simulink model "fw_rc_mapping"  (R2026b)
settings: Solver=VariableStepAuto
undefined symbols (not defined in the file or in its folder): P, Ts
libraries: simulink x27
settings Model: Creator=aomar  LastModifiedBy=aomar

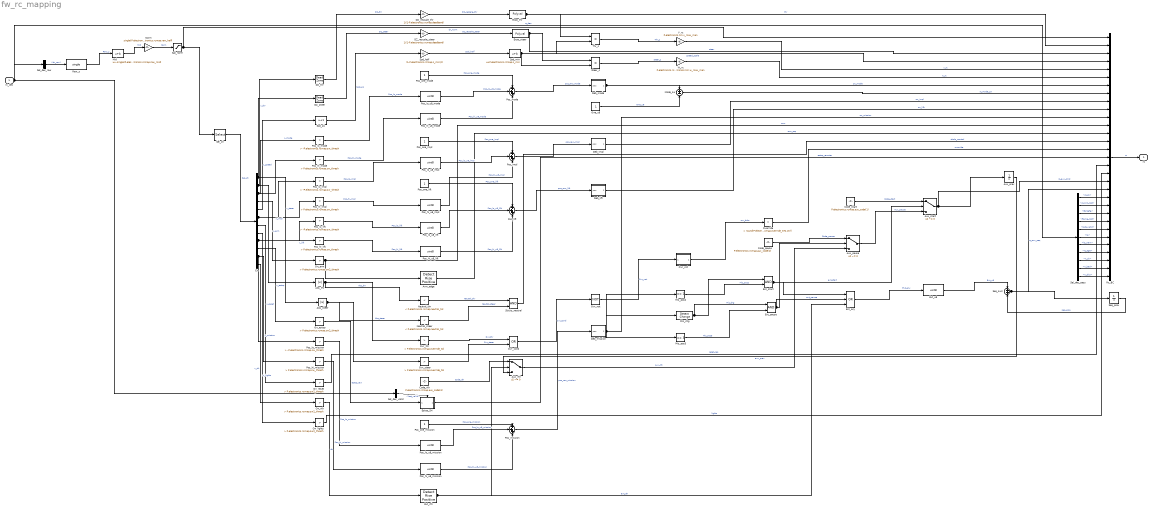
== system fw_rc_mapping ==
  rc_dec : Inport  SampleTime=Ts.ctrl
  Abs_steer : Abs  SaturateOnIntegerOverflow=off
  Abs_thr : Abs  SaturateOnIntegerOverflow=off
  Arm_edge : simulink/Logic and Bit Operations/Detect Rise Positive  vinit=0  OutDataTypeStr=boolean
  Aux_pause : Switch  Criteria=u2 ~= 0  SaturateOnIntegerOverflow=off  InputSameDT=off
  Aux_prev : UnitDelay  SampleTime=-1
  Aux_rth : Switch  Criteria=u2 ~= 0  SaturateOnIntegerOverflow=off  InputSameDT=off
  Aux_start : Switch  Criteria=u2 ~= 0  SaturateOnIntegerOverflow=off  InputSameDT=off
  Ch : Demux  Outputs=12
  Code_pause : Constant  Value=P.electronics.rcmap.aux_code(2)  OutDataTypeStr=uint8  SampleTime=-1
  Code_rth : Constant  Value=P.electronics.rcmap.aux_code(3)  OutDataTypeStr=uint8  SampleTime=-1
  Code_start : Constant  Value=P.electronics.rcmap.aux_code(1)  OutDataTypeStr=uint8  SampleTime=-1
  DZ_rescale_steer : Gain  Gain=1/(1-P.electronics.rcmap.deadband)
  DZ_rescale_thr : Gain  Gain=1/(1-P.electronics.rcmap.deadband)
  DZ_steer : DeadZone  LowerValue=-P.electronics.rcmap.deadband  UpperValue=P.electronics.rcmap.deadband
  DZ_thr : DeadZone  LowerValue=-P.electronics.rcmap.deadband  UpperValue=P.electronics.rcmap.deadband
  Deb_impl : Subsystem
  Deb_lift : Subsystem
  Deb_mission : Subsystem
  Deb_mode : Subsystem
  Estop_SH : Subsystem
  Evt_any : Logic  Operator=OR  Inputs=3  AllPortsSameDT=off  OutDataTypeStr=boolean
  Evt_pause : Logic  AllPortsSameDT=off  OutDataTypeStr=boolean
  Evt_rth : simulink/Logic and Bit Operations/Detect Rise Positive  vinit=0  OutDataTypeStr=boolean
  Evt_start : Logic  AllPortsSameDT=off  OutDataTypeStr=boolean
  Evt_u8 : DataTypeConversion  OutDataTypeStr=uint8  RndMeth=Round
  Expo_steer : Polyval  Coefs=[P.electronics.rcmap.expo_steer 0 1-P.electronics.rcmap.expo_steer 0]
  Expo_thr : Polyval  Coefs=[P.electronics.rcmap.expo_thr 0 1-P.electronics.rcmap.expo_thr 0]
  Mid : Bias  Bias=-single(P.electronics.rcmap.raw_mid)  SaturateOnIntegerOverflow=off
  Mis_chg : simulink/Logic and Bit Operations/Detect Change  vinit=P.electronics.rcmap.debounce_ic(4)  OutDataTypeStr=boolean
  Mis_pos2 : simulink/Logic and Bit Operations/Compare To Constant  relop===  const=2  OutDataTypeStr=boolean
  Mis_pos3 : simulink/Logic and Bit Operations/Compare To Constant  relop===  const=3  OutDataTypeStr=boolean
  Mode_sw : Sum  Inputs=+-  OutDataTypeStr=uint8
  Neutral_steer : simulink/Logic and Bit Operations/Compare To Constant  relop=<  const=P.electronics.rcmap.neutral_tol  OutDataTypeStr=boolean
  Neutral_thr : simulink/Logic and Bit Operations/Compare To Constant  relop=<  const=P.electronics.rcmap.neutral_tol  OutDataTypeStr=boolean
  Norm : Gain  Gain=single(P.electronics.rcmap.sign/P.electronics.rcmap.raw_half)
  On_arm : simulink/Logic and Bit Operations/Compare To Constant  relop=>  const=P.electronics.rcmap.sw2_thresh  OutDataTypeStr=boolean
  On_estop : simulink/Logic and Bit Operations/Compare To Constant  relop=>  const=P.electronics.rcmap.sw2_thresh  OutDataTypeStr=boolean
  On_lights : simulink/Logic and Bit Operations/Compare To Constant  relop=>  const=P.electronics.rcmap.sw2_thresh  OutDataTypeStr=boolean
  On_reset : simulink/Logic and Bit Operations/Compare To Constant  relop=>  const=P.electronics.rcmap.sw2_thresh  OutDataTypeStr=boolean
  On_rth : simulink/Logic and Bit Operations/Compare To Constant  relop=>  const=P.electronics.rcmap.sw2_thresh  OutDataTypeStr=boolean
  One_u8 : Constant  OutDataTypeStr=uint8  SampleTime=-1
  Override : simulink/Logic and Bit Operations/Compare To Constant  relop=>  const=round(P.electronics.rcmap.override_t/Ts.ctrl)  OutDataTypeStr=boolean
  Ovr_cnt : Subsystem
  Ovr_cond : Logic  Operator=OR  AllPortsSameDT=off  OutDataTypeStr=boolean
  Ovr_not : Logic  Operator=NOT  Inputs=1  AllPortsSameDT=off  OutDataTypeStr=boolean
  Ovr_steer : simulink/Logic and Bit Operations/Compare To Constant  relop=>  const=P.electronics.rcmap.override_tol  OutDataTypeStr=boolean
  Ovr_thr : simulink/Logic and Bit Operations/Compare To Constant  relop=>  const=P.electronics.rcmap.override_tol  OutDataTypeStr=boolean
  Pos_hi_impl : simulink/Logic and Bit Operations/Compare To Constant  relop=>  const=P.electronics.rcmap.sw_thresh  OutDataTypeStr=boolean
  Pos_hi_lift : simulink/Logic and Bit Operations/Compare To Constant  relop=>  const=P.electronics.rcmap.sw_thresh  OutDataTypeStr=boolean
  Pos_hi_mission : simulink/Logic and Bit Operations/Compare To Constant  relop=>  const=P.electronics.rcmap.sw_thresh  OutDataTypeStr=boolean
  Pos_hi_mode : simulink/Logic and Bit Operations/Compare To Constant  relop=>  const=P.electronics.rcmap.sw_thresh  OutDataTypeStr=boolean
  Pos_hi_u8_impl : DataTypeConversion  OutDataTypeStr=uint8  RndMeth=Round
  Pos_hi_u8_lift : DataTypeConversion  OutDataTypeStr=uint8  RndMeth=Round
  Pos_hi_u8_mission : DataTypeConversion  OutDataTypeStr=uint8  RndMeth=Round
  Pos_hi_u8_mode : DataTypeConversion  OutDataTypeStr=uint8  RndMeth=Round
  Pos_impl : Sum  Inputs=+++  OutDataTypeStr=uint8
  Pos_lift : Sum  Inputs=+++  OutDataTypeStr=uint8
  Pos_lo_impl : simulink/Logic and Bit Operations/Compare To Constant  relop=>  const=-P.electronics.rcmap.sw_thresh  OutDataTypeStr=boolean
  Pos_lo_lift : simulink/Logic and Bit Operations/Compare To Constant  relop=>  const=-P.electronics.rcmap.sw_thresh  OutDataTypeStr=boolean
  Pos_lo_mission : simulink/Logic and Bit Operations/Compare To Constant  relop=>  const=-P.electronics.rcmap.sw_thresh  OutDataTypeStr=boolean
  Pos_lo_mode : simulink/Logic and Bit Operations/Compare To Constant  relop=>  const=-P.electronics.rcmap.sw_thresh  OutDataTypeStr=boolean
  Pos_lo_u8_impl : DataTypeConversion  OutDataTypeStr=uint8  RndMeth=Round
  Pos_lo_u8_lift : DataTypeConversion  OutDataTypeStr=uint8  RndMeth=Round
  Pos_lo_u8_mission : DataTypeConversion  OutDataTypeStr=uint8  RndMeth=Round
  Pos_lo_u8_mode : DataTypeConversion  OutDataTypeStr=uint8  RndMeth=Round
  Pos_mission : Sum  Inputs=+++  OutDataTypeStr=uint8
  Pos_mode : Sum  Inputs=+++  OutDataTypeStr=uint8
  Pos_one_impl : Constant  OutDataTypeStr=uint8  SampleTime=-1
  Pos_one_lift : Constant  OutDataTypeStr=uint8  SampleTime=-1
  Pos_one_mission : Constant  OutDataTypeStr=uint8  SampleTime=-1
  Pos_one_mode : Constant  OutDataTypeStr=uint8  SampleTime=-1
  Raw_s : DataTypeConversion  OutDataTypeStr=single  RndMeth=Round
  Rc_BC : BusCreator  Inputs=31
  Sat_norm : Saturate  UpperLimit=1  LowerLimit=-1
  Sel_ch : Selector  InputPortWidth=16  IndexOptions=Index vector (dialog)  Indices=[P.electronics.rcmap.ch.steer P.electronics.rcmap.ch.thr P.electronics.rcmap.ch.mode P.electronics.rcmap.ch.arm P.electronics.rcmap.ch.speed P.electronics.rcmap.ch.impl P.electronics.rcmap.ch.reset P.electronics.rcmap.ch.lights P.electronics.rcmap.ch.lift P.electronics.rcmap.ch.estop P.electronics.rcmap.ch.mission P.electronics.rcmap.ch.rth]  OutputSizes=1
  Sel_dec_pass : BusSelector  OutputSignals=rc_ok,rc_link_lost,failsafe,frame_lost,last_valid,lq,lq_warn,rc_age,n_ok,n_bad,n_skip
  Sel_dec_raw : BusSelector  OutputSignals=ch_raw
  Sel_dec_valid : BusSelector  OutputSignals=last_valid
  Seq_prev : UnitDelay  SampleTime=-1
  Seq_sum : Sum  OutDataTypeStr=uint8
  Spd_half : Gain  Gain=(1-P.electronics.rcmap.s_min)/2
  Spd_min : Bias  Bias=P.electronics.rcmap.s_min  SaturateOnIntegerOverflow=off
  Spd_p1 : Bias  Bias=1  SaturateOnIntegerOverflow=off
  Steer_s : Product
  Sticks_neutral : Logic  AllPortsSameDT=off  OutDataTypeStr=boolean
  Thr_s : Product
  V_rc : Gain  Gain=P.electronics.lim.v_max_man
  W_rc : Gain  Gain=P.electronics.rcmap.steer_to_omega_sign*P.electronics.lim.w_max_man
  rc : Outport
  wires:
  rc_dec/1 -> Sel_dec_valid/1, Sel_dec_pass/1, Sel_dec_raw/1  "rc_dec"
  Sel_dec_raw/1 -> Raw_s/1  "<ch_raw>"
  Raw_s/1 -> Mid/1  "Raw_s"
  Mid/1 -> Norm/1  "Mid"
  Norm/1 -> Sat_norm/1  "Norm"
  Sat_norm/1 -> Sel_ch/1, Rc_BC/1  "ch_norm"
  Sel_ch/1 -> Ch/1  "Sel_ch"
  Ch/1 -> Abs_steer/1, DZ_steer/1  "x_steer"
  Ch/3 -> Pos_lo_mode/1, Pos_hi_mode/1  "x_mode"
  Ch/4 -> On_arm/1  "x_arm"
  Ch/5 -> Spd_p1/1  "x_speed"
  Ch/6 -> Pos_lo_impl/1, Pos_hi_impl/1  "x_impl"
  Ch/7 -> On_reset/1  "x_reset"
  Ch/8 -> On_lights/1  "x_lights"
  Ch/9 -> Pos_lo_lift/1, Pos_hi_lift/1  "x_lift"
  Ch/10 -> On_estop/1  "x_estop"
  Ch/12 -> On_rth/1  "x_rth"
  DZ_thr/1 -> DZ_rescale_thr/1  "DZ_thr"
  DZ_steer/1 -> DZ_rescale_steer/1  "DZ_steer"
  Pos_lo_mode/1 -> Pos_lo_u8_mode/1  "Pos_lo_mode"
  Pos_hi_mode/1 -> Pos_hi_u8_mode/1  "Pos_hi_mode"
  Pos_lo_impl/1 -> Pos_lo_u8_impl/1  "Pos_lo_impl"
  Pos_hi_impl/1 -> Pos_hi_u8_impl/1  "Pos_hi_impl"
  Pos_lo_lift/1 -> Pos_lo_u8_lift/1  "Pos_lo_lift"
  Pos_hi_lift/1 -> Pos_hi_u8_lift/1  "Pos_hi_lift"
  On_arm/1 -> Rc_BC/12, Arm_edge/1  "arm"
  Abs_thr/1 -> Ovr_thr/1, Neutral_thr/1  "Abs_thr"
  On_estop/1 -> Estop_SH/1(estop_raw)  "estop_raw"
  Pos_lo_mission/1 -> Pos_lo_u8_mission/1  "Pos_lo_mission"
  Pos_hi_mission/1 -> Pos_hi_u8_mission/1  "Pos_hi_mission"
  On_reset/1 -> Rc_BC/17  "reset_req"
  On_rth/1 -> Evt_rth/1  "rth"
  On_lights/1 -> Rc_BC/18  "lights"
  Spd_p1/1 -> Spd_half/1  "Spd_p1"
  Abs_steer/1 -> Ovr_steer/1, Neutral_steer/1  "Abs_steer"
  Sel_dec_valid/1 -> Estop_SH/Enable  "<last_valid>"
  DZ_rescale_thr/1 -> Expo_thr/1  "DZ_rescale_thr"
  DZ_rescale_steer/1 -> Expo_steer/1  "DZ_rescale_steer"
  Spd_half/1 -> Spd_min/1  "Spd_half"
  Pos_one_mode/1 -> Pos_mode/1  "Pos_one_mode"
  Pos_one_impl/1 -> Pos_impl/1  "Pos_one_impl"
  Pos_one_lift/1 -> Pos_lift/1  "Pos_one_lift"
  Neutral_thr/1 -> Sticks_neutral/1  "Neutral_thr"
  Neutral_steer/1 -> Sticks_neutral/2  "Neutral_steer"
  Ovr_thr/1 -> Ovr_cond/1  "Ovr_thr"
  Ovr_steer/1 -> Ovr_cond/2  "Ovr_steer"
  Code_rth/1 -> Aux_rth/1  "Code_rth"
  Pos_one_mission/1 -> Pos_mission/1  "Pos_one_mission"
  Estop_SH/1(estop_remote) -> Rc_BC/16  "estop_remote"
  Arm_edge/1 -> Rc_BC/13  "arm_req"
  Evt_rth/1 -> Evt_any/3, Aux_rth/2  "evt_rth"
  Pos_lo_u8_mode/1 -> Pos_mode/2  "Pos_lo_u8_mode"
  Pos_hi_u8_mode/1 -> Pos_mode/3  "Pos_hi_u8_mode"
  Pos_lo_u8_impl/1 -> Pos_impl/2  "Pos_lo_u8_impl"
  Pos_hi_u8_impl/1 -> Pos_impl/3  "Pos_hi_u8_impl"
  Pos_lo_u8_lift/1 -> Pos_lift/2  "Pos_lo_u8_lift"
  Pos_hi_u8_lift/1 -> Pos_lift/3  "Pos_hi_u8_lift"
  Pos_lo_u8_mission/1 -> Pos_mission/2  "Pos_lo_u8_mission"
  Pos_hi_u8_mission/1 -> Pos_mission/3  "Pos_hi_u8_mission"
  Pos_mode/1 -> Deb_mode/1(pos)  "pos_raw_mode"
  Pos_impl/1 -> Deb_impl/1(pos)  "pos_raw_impl"
  Pos_lift/1 -> Deb_lift/1(pos)  "pos_raw_lift"
  Pos_mission/1 -> Deb_mission/1(pos)  "pos_raw_mission"
  Sticks_neutral/1 -> Rc_BC/14  "sticks_neutral"
  Ovr_cond/1 -> Ovr_not/1  "ovr_cond"
  Spd_min/1 -> Thr_s/2, Steer_s/2, Rc_BC/4  "speed_scale"
  Aux_rth/1 -> Aux_pause/3  "Aux_rth"
  Expo_thr/1 -> Rc_BC/2, Thr_s/1  "thr"
  Expo_steer/1 -> Steer_s/1, Rc_BC/3  "steer"
  Thr_s/1 -> V_rc/1  "Thr_s"
  Steer_s/1 -> W_rc/1  "Steer_s"
  One_u8/1 -> Mode_sw/2  "One_u8"
  Ovr_not/1 -> Ovr_cnt/1(fresh)  "Ovr_not"
  Deb_mode/1(pos_deb) -> Mode_sw/1, Rc_BC/7  "sw_mode"
  Deb_impl/1(pos_deb) -> Rc_BC/9  "sw_impl"
  Deb_lift/1(pos_deb) -> Rc_BC/10  "sw_lift"
  Deb_mission/1(pos_deb) -> Rc_BC/11, Mis_pos2/1, Mis_chg/1, Mis_pos3/1  "sw_mission"
  Mode_sw/1 -> Rc_BC/8  "rc_mode_sw"
  V_rc/1 -> Rc_BC/5  "v_rc"
  W_rc/1 -> Rc_BC/6  "w_rc"
  Mis_pos2/1 -> Evt_start/2  "Mis_pos2"
  Mis_pos3/1 -> Evt_pause/2  "Mis_pos3"
  Ovr_cnt/1(ticks) -> Override/1  "ovr_ticks"
  Mis_chg/1 -> Evt_start/1, Evt_pause/1  "Mis_chg"
  Override/1 -> Rc_BC/15  "override"
  Code_pause/1 -> Aux_pause/1  "Code_pause"
  Evt_start/1 -> Aux_start/2, Evt_any/1  "evt_start"
  Evt_pause/1 -> Aux_pause/2, Evt_any/2  "evt_pause"
  Code_start/1 -> Aux_start/1  "Code_start"
  Evt_any/1 -> Evt_u8/1  "Evt_any"
  Aux_pause/1 -> Aux_start/3  "Aux_pause"
  Aux_start/1 -> Aux_prev/1, Rc_BC/19  "rc_aux_cmd"
  Evt_u8/1 -> Seq_sum/1  "Evt_u8"
  Seq_sum/1 -> Rc_BC/20, Seq_prev/1  "rc_aux_seq"
  Aux_prev/1 -> Aux_rth/3  "aux_prev"
  Sel_dec_pass/1 -> Rc_BC/21  "<rc_ok>"
  Sel_dec_pass/2 -> Rc_BC/22  "<rc_link_lost>"
  Sel_dec_pass/3 -> Rc_BC/23  "<failsafe>"
  Sel_dec_pass/4 -> Rc_BC/24  "<frame_lost>"
  Sel_dec_pass/5 -> Rc_BC/25  "<last_valid>"
  Sel_dec_pass/6 -> Rc_BC/26  "<lq>"
  Sel_dec_pass/7 -> Rc_BC/27  "<lq_warn>"
  Sel_dec_pass/8 -> Rc_BC/28  "<rc_age>"
  Sel_dec_pass/9 -> Rc_BC/29  "<n_ok>"
  Sel_dec_pass/10 -> Rc_BC/30  "<n_bad>"
  Sel_dec_pass/11 -> Rc_BC/31  "<n_skip>"
  Rc_BC/1 -> rc/1  "rc"
  Seq_prev/1 -> Seq_sum/2  "seq_prev"
  Ch/2 -> DZ_thr/1, Abs_thr/1  "x_thr"
  Ch/11 -> Pos_hi_mission/1, Pos_lo_mission/1  "x_mission"

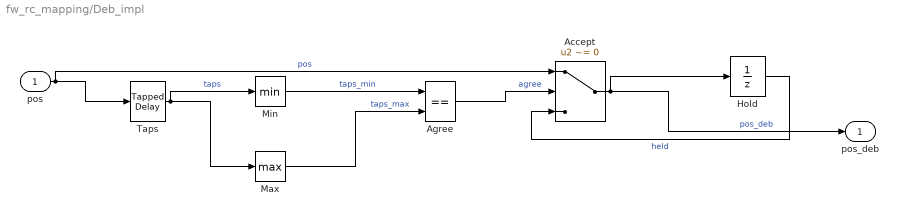
== system fw_rc_mapping/Deb_impl ==
  pos : Inport
  Accept : Switch  Criteria=u2 ~= 0  SaturateOnIntegerOverflow=off  InputSameDT=off
  Agree : RelationalOperator  Operator===  OutDataTypeStr=boolean  RndMeth=Simplest  InputSameDT=off
  Hold : UnitDelay  InitialCondition=P.electronics.rcmap.debounce_ic(2)  SampleTime=-1
  Max : MinMax  Function=max
  Min : MinMax
  Taps : simulink/Discrete/Tapped Delay  vinit=P.electronics.rcmap.debounce_ic(2)  samptime=-1  NumDelays=P.electronics.rcmap.debounce_n-1  DelayOrder=Oldest  includeCurrent=on
  pos_deb : Outport
  wires:
  pos/1 -> Taps/1, Accept/1  "pos"
  Taps/1 -> Max/1, Min/1  "taps"
  Min/1 -> Agree/1  "taps_min"
  Max/1 -> Agree/2  "taps_max"
  Agree/1 -> Accept/2  "agree"
  Accept/1 -> pos_deb/1, Hold/1  "pos_deb"
  Hold/1 -> Accept/3  "held"

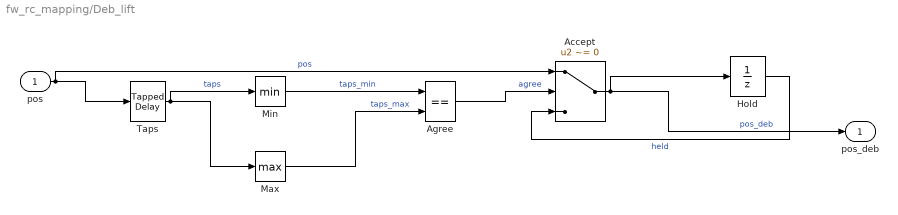
== system fw_rc_mapping/Deb_lift ==
  pos : Inport
  Accept : Switch  Criteria=u2 ~= 0  SaturateOnIntegerOverflow=off  InputSameDT=off
  Agree : RelationalOperator  Operator===  OutDataTypeStr=boolean  RndMeth=Simplest  InputSameDT=off
  Hold : UnitDelay  InitialCondition=P.electronics.rcmap.debounce_ic(3)  SampleTime=-1
  Max : MinMax  Function=max
  Min : MinMax
  Taps : simulink/Discrete/Tapped Delay  vinit=P.electronics.rcmap.debounce_ic(3)  samptime=-1  NumDelays=P.electronics.rcmap.debounce_n-1  DelayOrder=Oldest  includeCurrent=on
  pos_deb : Outport
  wires:
  pos/1 -> Taps/1, Accept/1  "pos"
  Taps/1 -> Max/1, Min/1  "taps"
  Min/1 -> Agree/1  "taps_min"
  Max/1 -> Agree/2  "taps_max"
  Agree/1 -> Accept/2  "agree"
  Accept/1 -> pos_deb/1, Hold/1  "pos_deb"
  Hold/1 -> Accept/3  "held"

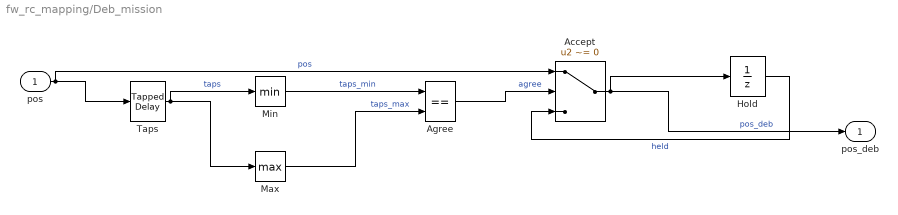
== system fw_rc_mapping/Deb_mission ==
  pos : Inport
  Accept : Switch  Criteria=u2 ~= 0  SaturateOnIntegerOverflow=off  InputSameDT=off
  Agree : RelationalOperator  Operator===  OutDataTypeStr=boolean  RndMeth=Simplest  InputSameDT=off
  Hold : UnitDelay  InitialCondition=P.electronics.rcmap.debounce_ic(4)  SampleTime=-1
  Max : MinMax  Function=max
  Min : MinMax
  Taps : simulink/Discrete/Tapped Delay  vinit=P.electronics.rcmap.debounce_ic(4)  samptime=-1  NumDelays=P.electronics.rcmap.debounce_n-1  DelayOrder=Oldest  includeCurrent=on
  pos_deb : Outport
  wires:
  pos/1 -> Taps/1, Accept/1  "pos"
  Taps/1 -> Max/1, Min/1  "taps"
  Min/1 -> Agree/1  "taps_min"
  Max/1 -> Agree/2  "taps_max"
  Agree/1 -> Accept/2  "agree"
  Accept/1 -> pos_deb/1, Hold/1  "pos_deb"
  Hold/1 -> Accept/3  "held"

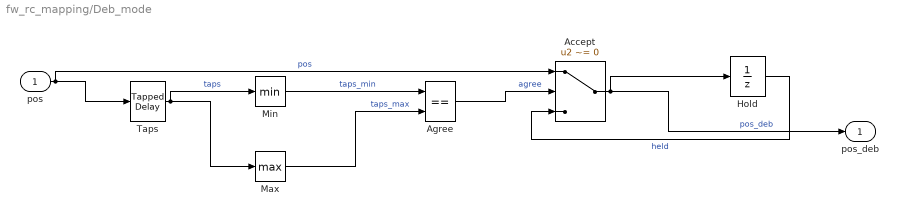
== system fw_rc_mapping/Deb_mode ==
  pos : Inport
  Accept : Switch  Criteria=u2 ~= 0  SaturateOnIntegerOverflow=off  InputSameDT=off
  Agree : RelationalOperator  Operator===  OutDataTypeStr=boolean  RndMeth=Simplest  InputSameDT=off
  Hold : UnitDelay  InitialCondition=P.electronics.rcmap.debounce_ic(1)  SampleTime=-1
  Max : MinMax  Function=max
  Min : MinMax
  Taps : simulink/Discrete/Tapped Delay  vinit=P.electronics.rcmap.debounce_ic(1)  samptime=-1  NumDelays=P.electronics.rcmap.debounce_n-1  DelayOrder=Oldest  includeCurrent=on
  pos_deb : Outport
  wires:
  pos/1 -> Taps/1, Accept/1  "pos"
  Taps/1 -> Max/1, Min/1  "taps"
  Min/1 -> Agree/1  "taps_min"
  Max/1 -> Agree/2  "taps_max"
  Agree/1 -> Accept/2  "agree"
  Accept/1 -> pos_deb/1, Hold/1  "pos_deb"
  Hold/1 -> Accept/3  "held"

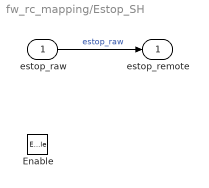
== system fw_rc_mapping/Estop_SH ==
  estop_raw : Inport
  Enable : EnablePort
  estop_remote : Outport  InitialOutput=false
  wires:
  estop_raw/1 -> estop_remote/1  "estop_raw"

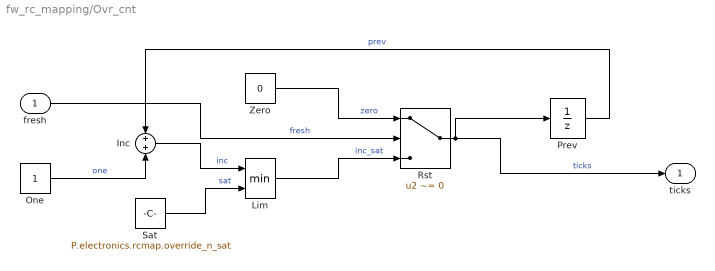
== system fw_rc_mapping/Ovr_cnt ==
  fresh : Inport
  Inc : Sum  OutDataTypeStr=uint16  SaturateOnIntegerOverflow=on
  Lim : MinMax  Inputs=2
  One : Constant  OutDataTypeStr=uint16  SampleTime=-1
  Prev : UnitDelay  SampleTime=-1
  Rst : Switch  Criteria=u2 ~= 0  SaturateOnIntegerOverflow=off  InputSameDT=off
  Sat : Constant  Value=P.electronics.rcmap.override_n_sat  OutDataTypeStr=uint16  SampleTime=-1
  Zero : Constant  Value=0  OutDataTypeStr=uint16  SampleTime=-1
  ticks : Outport
  wires:
  fresh/1 -> Rst/2  "fresh"
  One/1 -> Inc/2  "one"
  Inc/1 -> Lim/1  "inc"
  Sat/1 -> Lim/2  "sat"
  Zero/1 -> Rst/1  "zero"
  Lim/1 -> Rst/3  "inc_sat"
  Rst/1 -> ticks/1, Prev/1  "ticks"
  Prev/1 -> Inc/1  "prev"
